simulink model "phi4_m2_vr001_k5_3"  (R2026a)
settings: Solver=VariableStepAuto  StopTime=24.0
libraries: deeplib x1
settings Model: Creator=ldy  LastModifiedBy=harry_31916

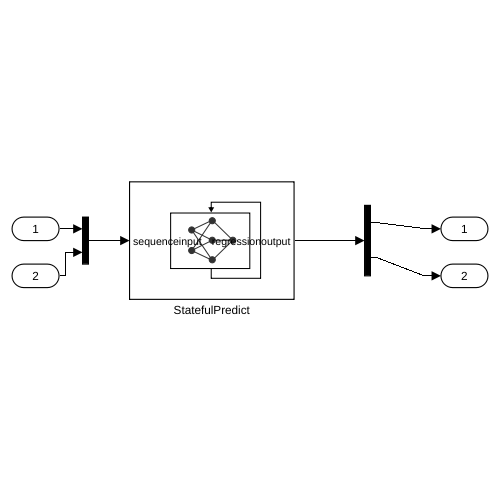
[thumbnail: Simulink's stored preview of the top-level diagram]
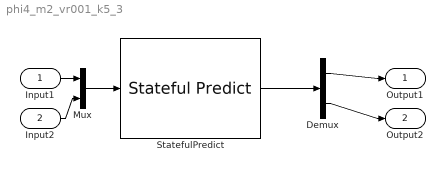
== system phi4_m2_vr001_k5_3 ==
  Input1 : Inport
  Input2 : Inport  Port=2
  Demux : Demux  Outputs=2
  Mux : Mux  Inputs=2
  StatefulPredict : deeplib/Stateful Predict  Network=Network from MAT-file  NetworkFunction=untitled  NetworkFilePath=phi4_m2_vr001_k5_3.mat  SimulateUsing=Auto mode  InputDataFormats={'',''}  SampleTime=1  ForceInterpretedSim=off  EnableDLNetwork=on  LastKnownNetworkFilePath=''  LastKnownNetworkTimeStamp=''
  Output1 : Outport
  Output2 : Outport  Port=2
  wires:
  Input1/1 -> Mux/1
  Input2/1 -> Mux/2
  Mux/1 -> StatefulPredict/1
  Demux/1 -> Output1/1
  Demux/2 -> Output2/1
  StatefulPredict/1 -> Demux/1
